simulink model "rg_pi_simple"  (R2025b)
settings: Solver=FixedStepDiscrete  StartTime=0  StopTime=240  FixedStep=1  RelTol=1e-3
PostLoadFcn:
  | addpath(fileparts(get_param(bdroot,'FileName')));
InitFcn:
  | addpath(fileparts(get_param(bdroot,'FileName'))); clear simple_mpct_step simple_rg_step;
model workspace (MAT data in the model file):
  reference_data.time = [0; 10; 80; 160; 240]
  reference_data.signals.values = [0; 0.7; 1.2; 0.3; 0.3]
  reference_data.signals.dimensions = 1
settings Model: Creator=alosw  LastModifiedBy=alosw
settings DataIOCC: SaveOutput=off  SignalLogging=off

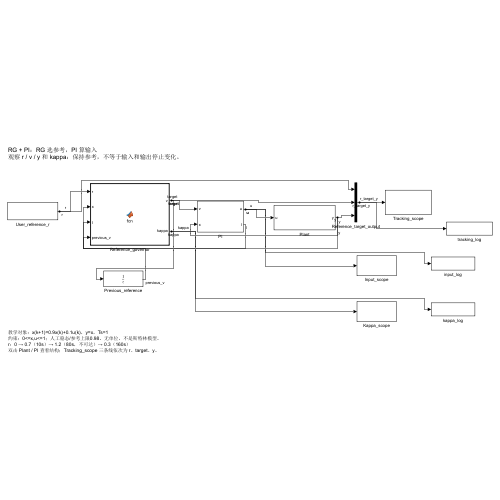
[thumbnail: Simulink's stored preview of the top-level diagram]
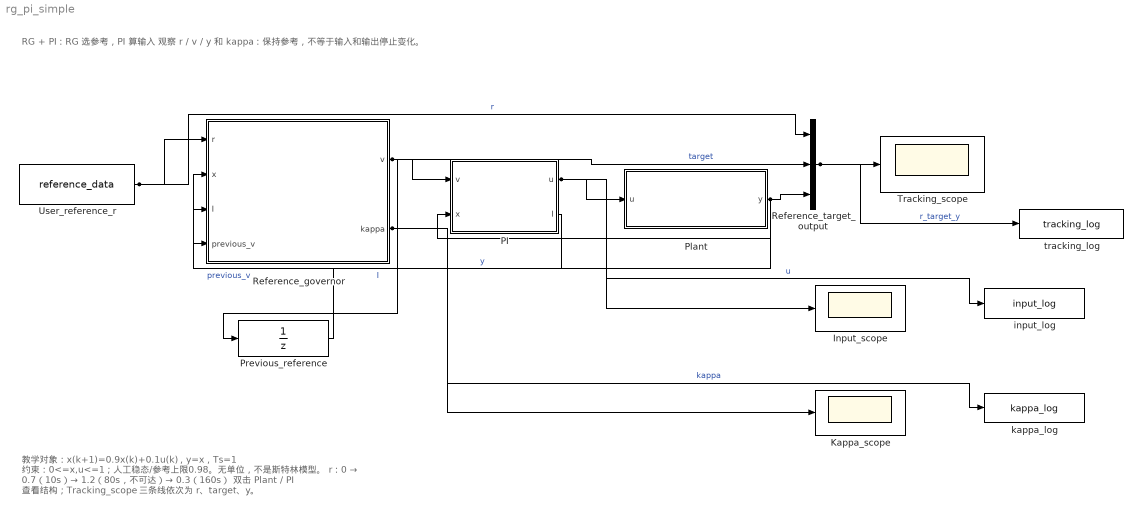
== system rg_pi_simple ==
  note: RG + PI：RG 选参考，PI 算输入
      | 观察 r / v / y 和 kappa：保持参考，不等于输入和输出停止变化。
  note: 教学对象：x(k+1)=0.9x(k)+0.1u(k)，y=x，Ts=1
      | 约束：0<=x,u<=1；人工稳态/参考上限0.98。无单位，不是斯特林模型。
      | r：0 → 0.7（10s）→ 1.2（80s，不可达）→ 0.3（160s）
      | 双击 Plant / PI 查看结构；Tracking_scope 三条线依次为 r、target、y。
  Input_scope : Scope
  Kappa_scope : Scope
  PI : Subsystem
  Plant : Subsystem
  Previous_reference : UnitDelay  HasFrameUpgradeWarning=on
  Reference_governor : MATLAB Function  TreatAsAtomicUnit=on
  Reference_target_output : Mux  Inputs=3
  Tracking_scope : Scope
  User_reference_r : FromWorkspace  VariableName=reference_data  SampleTime=1  Interpolate=off  OutputAfterFinalValue=Holding final value
  input_log : ToWorkspace  VariableName=input_log  SampleTime=-1
  kappa_log : ToWorkspace  VariableName=kappa_log  SampleTime=-1
  tracking_log : ToWorkspace  VariableName=tracking_log  SampleTime=-1
  wires:
  User_reference_r/1 -> Reference_governor/1(r), Reference_target_output/1  "r"
  Plant/1(y) -> Reference_governor/2(x), PI/2(x), Reference_target_output/3  "y"
  PI/2(I) -> Reference_governor/3(I)  "I"
  Previous_reference/1 -> Reference_governor/4(previous_v)  "previous_v"
  Reference_governor/1(v) -> Previous_reference/1, PI/1(v), Reference_target_output/2  "target"
  PI/1(u) -> Plant/1(u), Input_scope/1, input_log/1  "u"
  Reference_governor/2(kappa) -> Kappa_scope/1, kappa_log/1  "kappa"
  Reference_target_output/1 -> Tracking_scope/1, tracking_log/1  "r_target_y"

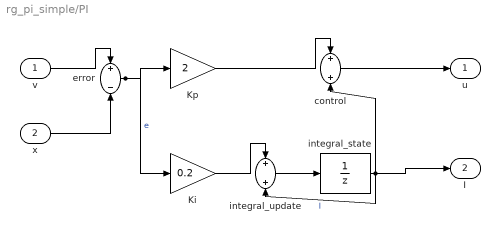
== system rg_pi_simple/PI ==
  v : Inport
  x : Inport  Port=2
  Ki : Gain  Gain=0.2
  Kp : Gain  Gain=2
  control : Sum
  error : Sum  Inputs=+-
  integral_state : UnitDelay  HasFrameUpgradeWarning=on
  integral_update : Sum
  u : Outport
  I : Outport  Port=2
  wires:
  v/1 -> error/1
  x/1 -> error/2
  error/1 -> Kp/1, Ki/1  "e"
  Kp/1 -> control/1
  Ki/1 -> integral_update/1
  integral_update/1 -> integral_state/1
  integral_state/1 -> integral_update/2, control/2, I/1  "I"
  control/1 -> u/1

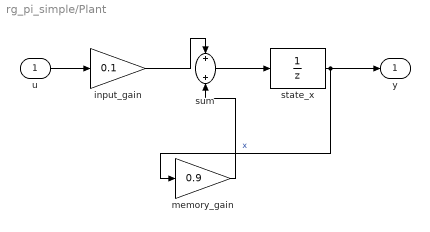
== system rg_pi_simple/Plant ==
  u : Inport
  input_gain : Gain  Gain=0.1
  memory_gain : Gain  Gain=0.9
  state_x : UnitDelay  HasFrameUpgradeWarning=on
  sum : Sum
  y : Outport
  wires:
  u/1 -> input_gain/1
  input_gain/1 -> sum/1
  sum/1 -> state_x/1
  state_x/1 -> y/1, memory_gain/1  "x"
  memory_gain/1 -> sum/2

== matlab function rg_pi_simple/Reference_governor ==
  data: r input; v output; x input; I input; previous_v input; kappa output
function [v,kappa] = fcn(r,x,I,previous_v)
% Predict the PI+plant closed loop, then maximize admissible kappa.
coder.extrinsic('simple_rg_step');
a=zeros(2,1);
a=simple_rg_step([r;x;I;previous_v]);
v=a(1);
kappa=a(2);
end
